simulink model "Sensores_Reales"  (R2026b)
settings: Solver=VariableStepAuto
values from neighbouring files (symbols this model uses):
  tau_RTD = 20    [coeficientes.m]
libraries: eeGeneralControl x5
settings Model: Creator=fedeb  LastModifiedBy=lamun

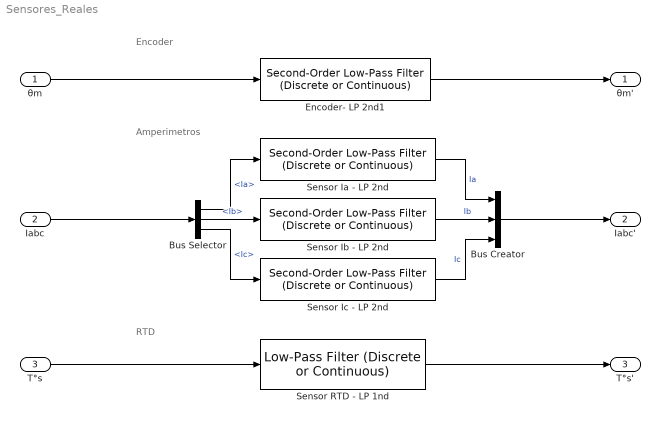
== system Sensores_Reales ==
  note: RTD
  note: Amperimetros
  note: Encoder
  θm : Inport
  Iabc : Inport  Port=2
  T°s : Inport  Port=3
  Bus Creator : BusCreator  Inputs=3
  Bus Selector : BusSelector  OutputSignals=Ia,Ib,Ic
  Encoder- LP 2nd1 : eeGeneralControl/Second-Order Low-Pass Filter (Discrete or Continuous)  A1=A1_E  A2=A2_E  init_option=Inherited from block input  x0=0  Ts=0
      settings: LibrarySourceBlock=|
      | ee_sl_lib/General Control/Second-Order
      | Low-Pass Filter
      | (Discrete or Continuous)
  Sensor Ia - LP 2nd : eeGeneralControl/Second-Order Low-Pass Filter (Discrete or Continuous)  A1=A1_I  A2=A2_I  init_option=Inherited from block input  x0=0  Ts=0
      settings: LibrarySourceBlock=|
      | ee_sl_lib/General Control/Second-Order
      | Low-Pass Filter
      | (Discrete or Continuous)
  Sensor Ib - LP 2nd : eeGeneralControl/Second-Order Low-Pass Filter (Discrete or Continuous)  A1=A1_I  A2=A2_I  init_option=Inherited from block input  x0=0  Ts=0
      settings: LibrarySourceBlock=|
      | ee_sl_lib/General Control/Second-Order
      | Low-Pass Filter
      | (Discrete or Continuous)
  Sensor Ic - LP 2nd : eeGeneralControl/Second-Order Low-Pass Filter (Discrete or Continuous)  A1=A1_I  A2=A2_I  init_option=Inherited from block input  x0=0  Ts=0
      settings: LibrarySourceBlock=|
      | ee_sl_lib/General Control/Second-Order
      | Low-Pass Filter
      | (Discrete or Continuous)
  Sensor RTD - LP 1nd : eeGeneralControl/Low-Pass Filter (Discrete or Continuous)  K=1  T=tau_RTD  B=inf  A=-inf  init_option=Inherited from block input  x0=0  Ts=0
  θm' : Outport
  Iabc' : Outport  Port=2
  T°s' : Outport  Port=3
  wires:
  Sensor Ic - LP 2nd/1 -> Bus Creator/3  "Ic"
  Sensor Ia - LP 2nd/1 -> Bus Creator/1  "Ia"
  Sensor Ib - LP 2nd/1 -> Bus Creator/2  "Ib"
  Bus Selector/3 -> Sensor Ic - LP 2nd/1  "<Ic>"
  Bus Selector/2 -> Sensor Ib - LP 2nd/1  "<Ib>"
  Bus Selector/1 -> Sensor Ia - LP 2nd/1  "<Ia>"
  Iabc/1 -> Bus Selector/1
  Bus Creator/1 -> Iabc'/1
  Sensor RTD - LP 1nd/1 -> T°s'/1
  T°s/1 -> Sensor RTD - LP 1nd/1
  Encoder- LP 2nd1/1 -> θm'/1
  θm/1 -> Encoder- LP 2nd1/1
